simulink model "Battery_ConstT_Lumped"  (R2026b)
settings: Solver=VariableStepAuto
undefined symbols (not defined in the file or in its folder): battery_builder_rtmsupport, gcbh, Vehicle
libraries: Battery_ConstT_Lumped_lib x10
settings Model: Creator=andrei  LastModifiedBy=andrei

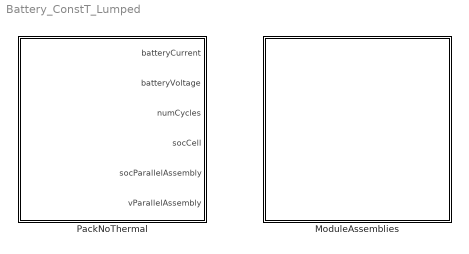
== system Battery_ConstT_Lumped ==
  ModuleAssemblies : Subsystem
  PackNoThermal : Subsystem  LoadFcn=battery_builder_rtmsupport('loadfcn',gcbh);  mask{BatteryPack=Vehicle.Powertrain.Power.Battery.BatteryPack}
      mask prompts: BatteryPack "Cell parameter structure (single-cell values)"
      mask help: Constant-temperature battery pack: 75 cells in series and 5 in parallel. Supply single-cell capacity (Ah), open-circuit voltage (V), resistance (Ohm), voltage limits, SOC and temperature lookup data. Series/parallel scaling is performed internally by the lumping adapters. Each module has one scalar representative-cell state.
      settings: CopyFcn=battery_builder_rtmsupport('copyfcn',gcbh);  PreCopyFcn=battery_builder_rtmsupport('precopyfcn',gcbh);  PreDeleteFcn=battery_builder_rtmsupport('predeletefcn',gcbh);  PortSchema="{\"entries\":[{\"content\":{\"sides\":[{\"content\":{\"connectorIds\":[\"LConn1\"]},\"type\":\"ConnectorPlacement.EquallySpacedRectSide\",\"uuid\":\"573f1e22-4fbd-4738-9df4-0664fa5945b1\"},{\"content\":{\"connectorIds\":[\"RConn1\"],\"side\":\"RIGHT\"},\"type\":\"ConnectorPlacement.EquallySpacedRectSide\",\"uuid\":\"3b7d0607-87fd-441c-83fa-686a76e2ac3c\"},{\"content\":{\"side\":\"TOP\"},\"type\":\"ConnectorPlacement.EquallySpacedRectSide\",\"uuid\":\"c7cf6d18-6b66-4f32-bb78-2b2f851634dd\"},{\"content\":{\"connectorIds\":[\"Out1\",\"Out2\",\"Out3\",\"Out4\",\"Out5\",\"Out6\"],\"side\":\"BOTTOM\"},\"type\":\"ConnectorPlacement.EquallySpacedRectSide\",\"uuid\":\"e3b01d7d-4c21-4d45-a142-ed30dadf23ae\"}]},\"type\":\"ConnectorPlacement.EquallySpacedConnector\",\"uuid\":\"ee102ac4-66a3-49fe-a4f4-6ac82dff7d13\"}],\"packageUris\":[\"http://schema.mathworks.com/mf0/Connector/R2020b\"],\"version\":\"1.0\"}"
      mask Display: image('$imagefile')

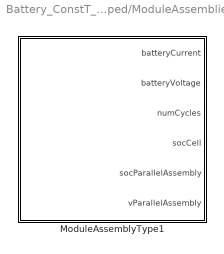
== system Battery_ConstT_Lumped/ModuleAssemblies ==
  ModuleAssemblyType1 : Subsystem  LoadFcn=battery_builder_rtmsupport('loadfcn',gcbh);
      settings: CopyFcn=battery_builder_rtmsupport('copyfcn',gcbh);  PreCopyFcn=battery_builder_rtmsupport('precopyfcn',gcbh);  PreDeleteFcn=battery_builder_rtmsupport('predeletefcn',gcbh);  PortSchema="{\"entries\":[{\"content\":{\"sides\":[{\"content\":{\"connectorIds\":[\"LConn1\"]},\"type\":\"ConnectorPlacement.EquallySpacedRectSide\",\"uuid\":\"573f1e22-4fbd-4738-9df4-0664fa5945b1\"},{\"content\":{\"connectorIds\":[\"RConn1\"],\"side\":\"RIGHT\"},\"type\":\"ConnectorPlacement.EquallySpacedRectSide\",\"uuid\":\"3b7d0607-87fd-441c-83fa-686a76e2ac3c\"},{\"content\":{\"side\":\"TOP\"},\"type\":\"ConnectorPlacement.EquallySpacedRectSide\",\"uuid\":\"c7cf6d18-6b66-4f32-bb78-2b2f851634dd\"},{\"content\":{\"connectorIds\":[\"Out1\",\"Out2\",\"Out3\",\"Out4\",\"Out5\",\"Out6\"],\"side\":\"BOTTOM\"},\"type\":\"ConnectorPlacement.EquallySpacedRectSide\",\"uuid\":\"1d9f9d4f-5931-4e62-be25-ddff82a8678d\"}]},\"type\":\"ConnectorPlacement.EquallySpacedConnector\",\"uuid\":\"ee102ac4-66a3-49fe-a4f4-6ac82dff7d13\"}],\"packageUris\":[\"http://schema.mathworks.com/mf0/Connector/R2020b\"],\"version\":\"1.0\"}"
      mask Display: image('$imagefile')

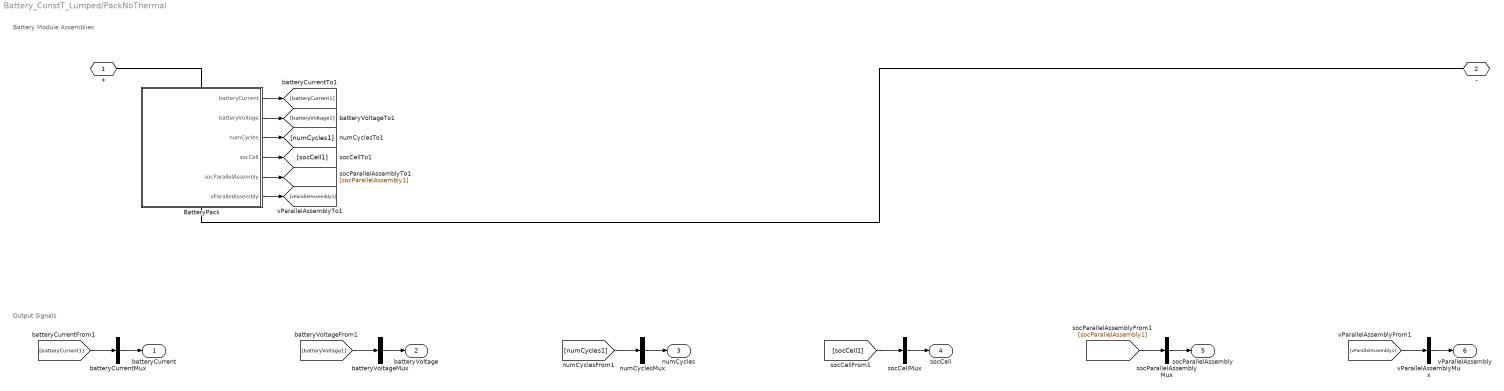
== system Battery_ConstT_Lumped/PackNoThermal ==
  note: Battery Module Assemblies
  note: Output Signals
  BatteryPack : Subsystem  LoadFcn=battery_builder_rtmsupport('loadfcn',gcbh);
      settings: CopyFcn=battery_builder_rtmsupport('copyfcn',gcbh);  PreCopyFcn=battery_builder_rtmsupport('precopyfcn',gcbh);  PreDeleteFcn=battery_builder_rtmsupport('predeletefcn',gcbh);  PortSchema="{\"entries\":[{\"content\":{\"sides\":[{\"content\":{\"connectorIds\":[\"LConn1\"]},\"type\":\"ConnectorPlacement.EquallySpacedRectSide\",\"uuid\":\"573f1e22-4fbd-4738-9df4-0664fa5945b1\"},{\"content\":{\"connectorIds\":[\"RConn1\"],\"side\":\"RIGHT\"},\"type\":\"ConnectorPlacement.EquallySpacedRectSide\",\"uuid\":\"3b7d0607-87fd-441c-83fa-686a76e2ac3c\"},{\"content\":{\"side\":\"TOP\"},\"type\":\"ConnectorPlacement.EquallySpacedRectSide\",\"uuid\":\"c7cf6d18-6b66-4f32-bb78-2b2f851634dd\"},{\"content\":{\"connectorIds\":[\"Out1\",\"Out2\",\"Out3\",\"Out4\",\"Out5\",\"Out6\"],\"side\":\"BOTTOM\"},\"type\":\"ConnectorPlacement.EquallySpacedRectSide\",\"uuid\":\"1d9f9d4f-5931-4e62-be25-ddff82a8678d\"}]},\"type\":\"ConnectorPlacement.EquallySpacedConnector\",\"uuid\":\"ee102ac4-66a3-49fe-a4f4-6ac82dff7d13\"}],\"packageUris\":[\"http://schema.mathworks.com/mf0/Connector/R2020b\"],\"version\":\"1.0\"}"
      mask Display: image('$imagefile')
  batteryCurrentMux : Mux  Inputs=1
  batteryVoltageMux : Mux  Inputs=1
  numCyclesMux : Mux  Inputs=1
  socCellMux : Mux  Inputs=1
  socParallelAssemblyMux : Mux  Inputs=1
  vParallelAssemblyMux : Mux  Inputs=1
  + : PMIOPort  Side=Left
  - : PMIOPort  Port=2  Side=Right
  batteryCurrent : Outport
  batteryVoltage : Outport  Port=2
  numCycles : Outport  Port=3
  socCell : Outport  Port=4
  socParallelAssembly : Outport  Port=5
  vParallelAssembly : Outport  Port=6
  wires:
  BatteryPack/1(batteryCurrent) -> [batteryCurrent1]
  batteryCurrentMux/1 -> batteryCurrent/1
  [batteryCurrent1] -> batteryCurrentMux/1
  BatteryPack/2(batteryVoltage) -> [batteryVoltage1]
  batteryVoltageMux/1 -> batteryVoltage/1
  [batteryVoltage1] -> batteryVoltageMux/1
  BatteryPack/3(numCycles) -> [numCycles1]
  numCyclesMux/1 -> numCycles/1
  [numCycles1] -> numCyclesMux/1
  BatteryPack/4(socCell) -> [socCell1]
  socCellMux/1 -> socCell/1
  [socCell1] -> socCellMux/1
  BatteryPack/5(socParallelAssembly) -> [socParallelAssembly1]
  socParallelAssemblyMux/1 -> socParallelAssembly/1
  [socParallelAssembly1] -> socParallelAssemblyMux/1
  BatteryPack/6(vParallelAssembly) -> [vParallelAssembly1]
  vParallelAssemblyMux/1 -> vParallelAssembly/1
  [vParallelAssembly1] -> vParallelAssemblyMux/1
  connections:
  BatteryPack/LConn1 -- +/RConn1
  BatteryPack/RConn1 -- -/RConn1

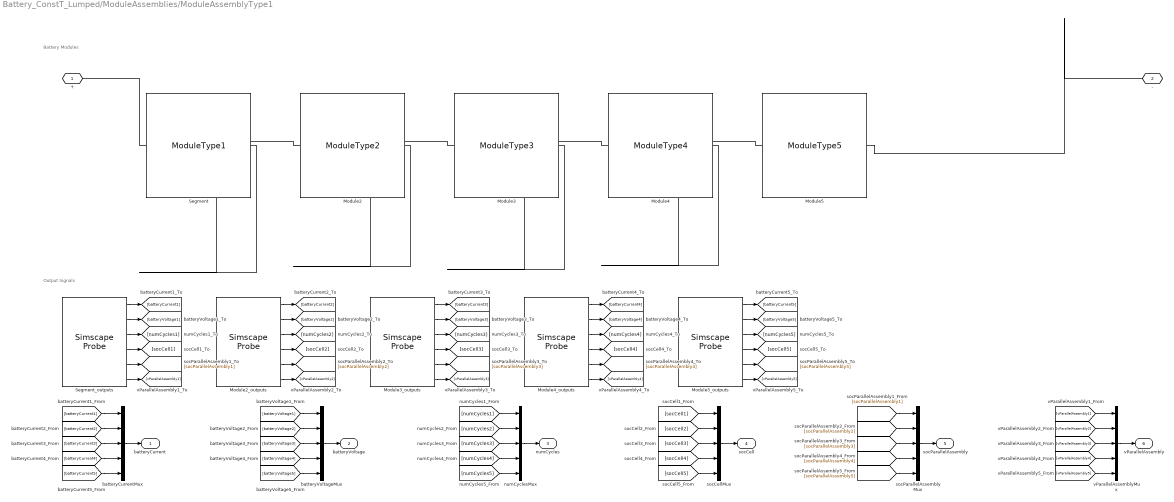
== system Battery_ConstT_Lumped/ModuleAssemblies/ModuleAssemblyType1 ==
  note: Battery Modules
  note: Output Signals
  Module2 : Battery_ConstT_Lumped_lib/Modules/ModuleType2  BatteryCapacityCell=27 A*hr  ExtrapolationMethodCell=simscape.enum.extrapolation.nearest  SOCBreakpointsCell=[0, .1, .25, .5, .75, .9, 1]  TemperatureBreakpointsCell=[278, 293, 313] K  OpenCircuitVoltageThermalCell=[3.49, 3.5, 3.51; 3.55, 3.57, 3.56; 3.62, 3.63, 3.64; 3.71, 3.71, 3.72; 3.91, 3.93, 3.94; 4.07, 4.08, 4.08; 4.19, 4.19, 4.19] V  VoltageRangeCell=[0, inf] V  ResistanceSOCBreakpointsCell=[0, .1, .25, .5, .75, .9, 1]  ResistanceTemperatureBreakpointsCell=[278, 293, 313] K  R0ThermalCell=[.0117, .0085, .009; .011, .0085, .009; .0114, .0087, .0092; .0107, .0082, .0088; .0107, .0083, .0091; .0113, .0085, .0089; .0116, .0085, .0089] Ohm  SimulationTemperatureCell=298.15 K  socCell_specify=off  socCell_priority=High  socCell=1  socCell_nominal_specify=off  socCell_nominal_value=1  socCell_nominal_unit=1  batteryVoltage_specify=off  batteryVoltage_priority=None  batteryVoltage=0 V  batteryVoltage_nominal_specify=off  batteryVoltage_nominal_value=1  batteryVoltage_nominal_unit=V  batteryCurrent_specify=off  batteryCurrent_priority=None  batteryCurrent=0 A  batteryCurrent_nominal_specify=off  batteryCurrent_nominal_value=1  batteryCurrent_nominal_unit=A  numCycles_specify=off  numCycles_priority=High  numCycles=0  numCycles_nominal_specify=off  numCycles_nominal_value=1  numCycles_nominal_unit=1  vParallelAssembly_specify=off  vParallelAssembly_priority=None  vParallelAssembly=repmat(0, 15, 1) V  vParallelAssembly_nominal_specify=off  vParallelAssembly_nominal_value=1  vParallelAssembly_nominal_unit=V  socParallelAssembly_specify=off  socParallelAssembly_priority=None  socParallelAssembly=repmat(1, 15, 1)  socParallelAssembly_nominal_specify=off  socParallelAssembly_nominal_value=1  socParallelAssembly_nominal_unit=1
  Module2_outputs : SimscapeProbe  BoundBlock=4  Variables="{\"batteryCurrent\":{\"Probing\":\"ON\"},\"batteryVoltage\":{\"Probing\":\"ON\"},\"numCycles\":{\"Probing\":\"ON\"},\"socCell\":{\"Probing\":\"ON\"},\"socParallelAssembly\":{\"Probing\":\"ON\"},\"vParallelAssembly\":{\"Probing\":\"ON\"}}"
  Module3 : Battery_ConstT_Lumped_lib/Modules/ModuleType3  BatteryCapacityCell=27 A*hr  ExtrapolationMethodCell=simscape.enum.extrapolation.nearest  SOCBreakpointsCell=[0, .1, .25, .5, .75, .9, 1]  TemperatureBreakpointsCell=[278, 293, 313] K  OpenCircuitVoltageThermalCell=[3.49, 3.5, 3.51; 3.55, 3.57, 3.56; 3.62, 3.63, 3.64; 3.71, 3.71, 3.72; 3.91, 3.93, 3.94; 4.07, 4.08, 4.08; 4.19, 4.19, 4.19] V  VoltageRangeCell=[0, inf] V  ResistanceSOCBreakpointsCell=[0, .1, .25, .5, .75, .9, 1]  ResistanceTemperatureBreakpointsCell=[278, 293, 313] K  R0ThermalCell=[.0117, .0085, .009; .011, .0085, .009; .0114, .0087, .0092; .0107, .0082, .0088; .0107, .0083, .0091; .0113, .0085, .0089; .0116, .0085, .0089] Ohm  SimulationTemperatureCell=298.15 K  socCell_specify=off  socCell_priority=High  socCell=1  socCell_nominal_specify=off  socCell_nominal_value=1  socCell_nominal_unit=1  batteryVoltage_specify=off  batteryVoltage_priority=None  batteryVoltage=0 V  batteryVoltage_nominal_specify=off  batteryVoltage_nominal_value=1  batteryVoltage_nominal_unit=V  batteryCurrent_specify=off  batteryCurrent_priority=None  batteryCurrent=0 A  batteryCurrent_nominal_specify=off  batteryCurrent_nominal_value=1  batteryCurrent_nominal_unit=A  numCycles_specify=off  numCycles_priority=High  numCycles=0  numCycles_nominal_specify=off  numCycles_nominal_value=1  numCycles_nominal_unit=1  vParallelAssembly_specify=off  vParallelAssembly_priority=None  vParallelAssembly=repmat(0, 15, 1) V  vParallelAssembly_nominal_specify=off  vParallelAssembly_nominal_value=1  vParallelAssembly_nominal_unit=V  socParallelAssembly_specify=off  socParallelAssembly_priority=None  socParallelAssembly=repmat(1, 15, 1)  socParallelAssembly_nominal_specify=off  socParallelAssembly_nominal_value=1  socParallelAssembly_nominal_unit=1
  Module3_outputs : SimscapeProbe  BoundBlock=5  Variables="{\"batteryCurrent\":{\"Probing\":\"ON\"},\"batteryVoltage\":{\"Probing\":\"ON\"},\"numCycles\":{\"Probing\":\"ON\"},\"socCell\":{\"Probing\":\"ON\"},\"socParallelAssembly\":{\"Probing\":\"ON\"},\"vParallelAssembly\":{\"Probing\":\"ON\"}}"
  Module4 : Battery_ConstT_Lumped_lib/Modules/ModuleType4  BatteryCapacityCell=27 A*hr  ExtrapolationMethodCell=simscape.enum.extrapolation.nearest  SOCBreakpointsCell=[0, .1, .25, .5, .75, .9, 1]  TemperatureBreakpointsCell=[278, 293, 313] K  OpenCircuitVoltageThermalCell=[3.49, 3.5, 3.51; 3.55, 3.57, 3.56; 3.62, 3.63, 3.64; 3.71, 3.71, 3.72; 3.91, 3.93, 3.94; 4.07, 4.08, 4.08; 4.19, 4.19, 4.19] V  VoltageRangeCell=[0, inf] V  ResistanceSOCBreakpointsCell=[0, .1, .25, .5, .75, .9, 1]  ResistanceTemperatureBreakpointsCell=[278, 293, 313] K  R0ThermalCell=[.0117, .0085, .009; .011, .0085, .009; .0114, .0087, .0092; .0107, .0082, .0088; .0107, .0083, .0091; .0113, .0085, .0089; .0116, .0085, .0089] Ohm  SimulationTemperatureCell=298.15 K  socCell_specify=off  socCell_priority=High  socCell=1  socCell_nominal_specify=off  socCell_nominal_value=1  socCell_nominal_unit=1  batteryVoltage_specify=off  batteryVoltage_priority=None  batteryVoltage=0 V  batteryVoltage_nominal_specify=off  batteryVoltage_nominal_value=1  batteryVoltage_nominal_unit=V  batteryCurrent_specify=off  batteryCurrent_priority=None  batteryCurrent=0 A  batteryCurrent_nominal_specify=off  batteryCurrent_nominal_value=1  batteryCurrent_nominal_unit=A  numCycles_specify=off  numCycles_priority=High  numCycles=0  numCycles_nominal_specify=off  numCycles_nominal_value=1  numCycles_nominal_unit=1  vParallelAssembly_specify=off  vParallelAssembly_priority=None  vParallelAssembly=repmat(0, 15, 1) V  vParallelAssembly_nominal_specify=off  vParallelAssembly_nominal_value=1  vParallelAssembly_nominal_unit=V  socParallelAssembly_specify=off  socParallelAssembly_priority=None  socParallelAssembly=repmat(1, 15, 1)  socParallelAssembly_nominal_specify=off  socParallelAssembly_nominal_value=1  socParallelAssembly_nominal_unit=1
  Module4_outputs : SimscapeProbe  BoundBlock=6  Variables="{\"batteryCurrent\":{\"Probing\":\"ON\"},\"batteryVoltage\":{\"Probing\":\"ON\"},\"numCycles\":{\"Probing\":\"ON\"},\"socCell\":{\"Probing\":\"ON\"},\"socParallelAssembly\":{\"Probing\":\"ON\"},\"vParallelAssembly\":{\"Probing\":\"ON\"}}"
  Module5 : Battery_ConstT_Lumped_lib/Modules/ModuleType5  BatteryCapacityCell=27 A*hr  ExtrapolationMethodCell=simscape.enum.extrapolation.nearest  SOCBreakpointsCell=[0, .1, .25, .5, .75, .9, 1]  TemperatureBreakpointsCell=[278, 293, 313] K  OpenCircuitVoltageThermalCell=[3.49, 3.5, 3.51; 3.55, 3.57, 3.56; 3.62, 3.63, 3.64; 3.71, 3.71, 3.72; 3.91, 3.93, 3.94; 4.07, 4.08, 4.08; 4.19, 4.19, 4.19] V  VoltageRangeCell=[0, inf] V  ResistanceSOCBreakpointsCell=[0, .1, .25, .5, .75, .9, 1]  ResistanceTemperatureBreakpointsCell=[278, 293, 313] K  R0ThermalCell=[.0117, .0085, .009; .011, .0085, .009; .0114, .0087, .0092; .0107, .0082, .0088; .0107, .0083, .0091; .0113, .0085, .0089; .0116, .0085, .0089] Ohm  SimulationTemperatureCell=298.15 K  socCell_specify=off  socCell_priority=High  socCell=1  socCell_nominal_specify=off  socCell_nominal_value=1  socCell_nominal_unit=1  batteryVoltage_specify=off  batteryVoltage_priority=None  batteryVoltage=0 V  batteryVoltage_nominal_specify=off  batteryVoltage_nominal_value=1  batteryVoltage_nominal_unit=V  batteryCurrent_specify=off  batteryCurrent_priority=None  batteryCurrent=0 A  batteryCurrent_nominal_specify=off  batteryCurrent_nominal_value=1  batteryCurrent_nominal_unit=A  numCycles_specify=off  numCycles_priority=High  numCycles=0  numCycles_nominal_specify=off  numCycles_nominal_value=1  numCycles_nominal_unit=1  vParallelAssembly_specify=off  vParallelAssembly_priority=None  vParallelAssembly=repmat(0, 15, 1) V  vParallelAssembly_nominal_specify=off  vParallelAssembly_nominal_value=1  vParallelAssembly_nominal_unit=V  socParallelAssembly_specify=off  socParallelAssembly_priority=None  socParallelAssembly=repmat(1, 15, 1)  socParallelAssembly_nominal_specify=off  socParallelAssembly_nominal_value=1  socParallelAssembly_nominal_unit=1
  Module5_outputs : SimscapeProbe  BoundBlock=7  Variables="{\"batteryCurrent\":{\"Probing\":\"ON\"},\"batteryVoltage\":{\"Probing\":\"ON\"},\"numCycles\":{\"Probing\":\"ON\"},\"socCell\":{\"Probing\":\"ON\"},\"socParallelAssembly\":{\"Probing\":\"ON\"},\"vParallelAssembly\":{\"Probing\":\"ON\"}}"
  Segment : Battery_ConstT_Lumped_lib/Modules/ModuleType1  BatteryCapacityCell=27 A*hr  ExtrapolationMethodCell=simscape.enum.extrapolation.nearest  SOCBreakpointsCell=[0, .1, .25, .5, .75, .9, 1]  TemperatureBreakpointsCell=[278, 293, 313] K  OpenCircuitVoltageThermalCell=[3.49, 3.5, 3.51; 3.55, 3.57, 3.56; 3.62, 3.63, 3.64; 3.71, 3.71, 3.72; 3.91, 3.93, 3.94; 4.07, 4.08, 4.08; 4.19, 4.19, 4.19] V  VoltageRangeCell=[0, inf] V  ResistanceSOCBreakpointsCell=[0, .1, .25, .5, .75, .9, 1]  ResistanceTemperatureBreakpointsCell=[278, 293, 313] K  R0ThermalCell=[.0117, .0085, .009; .011, .0085, .009; .0114, .0087, .0092; .0107, .0082, .0088; .0107, .0083, .0091; .0113, .0085, .0089; .0116, .0085, .0089] Ohm  SimulationTemperatureCell=298.15 K  socCell_specify=off  socCell_priority=High  socCell=1  socCell_nominal_specify=off  socCell_nominal_value=1  socCell_nominal_unit=1  batteryVoltage_specify=off  batteryVoltage_priority=None  batteryVoltage=0 V  batteryVoltage_nominal_specify=off  batteryVoltage_nominal_value=1  batteryVoltage_nominal_unit=V  batteryCurrent_specify=off  batteryCurrent_priority=None  batteryCurrent=0 A  batteryCurrent_nominal_specify=off  batteryCurrent_nominal_value=1  batteryCurrent_nominal_unit=A  numCycles_specify=off  numCycles_priority=High  numCycles=0  numCycles_nominal_specify=off  numCycles_nominal_value=1  numCycles_nominal_unit=1  vParallelAssembly_specify=off  vParallelAssembly_priority=None  vParallelAssembly=repmat(0, 15, 1) V  vParallelAssembly_nominal_specify=off  vParallelAssembly_nominal_value=1  vParallelAssembly_nominal_unit=V  socParallelAssembly_specify=off  socParallelAssembly_priority=None  socParallelAssembly=repmat(1, 15, 1)  socParallelAssembly_nominal_specify=off  socParallelAssembly_nominal_value=1  socParallelAssembly_nominal_unit=1
  Segment_outputs : SimscapeProbe  BoundBlock=3  Variables="{\"batteryCurrent\":{\"Probing\":\"ON\"},\"batteryVoltage\":{\"Probing\":\"ON\"},\"numCycles\":{\"Probing\":\"ON\"},\"socCell\":{\"Probing\":\"ON\"},\"socParallelAssembly\":{\"Probing\":\"ON\"},\"vParallelAssembly\":{\"Probing\":\"ON\"}}"
  batteryCurrentMux : Mux  Inputs=5
  batteryVoltageMux : Mux  Inputs=5
  numCyclesMux : Mux  Inputs=5
  socCellMux : Mux  Inputs=5
  socParallelAssemblyMux : Mux  Inputs=5
  vParallelAssemblyMux : Mux  Inputs=5
  + : PMIOPort  Side=Left
  - : PMIOPort  Port=2  Side=Right
  batteryCurrent : Outport
  batteryVoltage : Outport  Port=2
  numCycles : Outport  Port=3
  socCell : Outport  Port=4
  socParallelAssembly : Outport  Port=5
  vParallelAssembly : Outport  Port=6
  wires:
  Segment_outputs/1 -> [batteryCurrent1]
  batteryCurrentMux/1 -> batteryCurrent/1
  [batteryCurrent1] -> batteryCurrentMux/1
  Segment_outputs/2 -> [batteryVoltage1]
  batteryVoltageMux/1 -> batteryVoltage/1
  [batteryVoltage1] -> batteryVoltageMux/1
  Segment_outputs/3 -> [numCycles1]
  numCyclesMux/1 -> numCycles/1
  [numCycles1] -> numCyclesMux/1
  Segment_outputs/4 -> [socCell1]
  socCellMux/1 -> socCell/1
  [socCell1] -> socCellMux/1
  Segment_outputs/5 -> [socParallelAssembly1]
  socParallelAssemblyMux/1 -> socParallelAssembly/1
  [socParallelAssembly1] -> socParallelAssemblyMux/1
  Segment_outputs/6 -> [vParallelAssembly1]
  vParallelAssemblyMux/1 -> vParallelAssembly/1
  [vParallelAssembly1] -> vParallelAssemblyMux/1
  Module2_outputs/1 -> [batteryCurrent2]
  [batteryCurrent2] -> batteryCurrentMux/2
  Module2_outputs/2 -> [batteryVoltage2]
  [batteryVoltage2] -> batteryVoltageMux/2
  Module2_outputs/3 -> [numCycles2]
  [numCycles2] -> numCyclesMux/2
  Module2_outputs/4 -> [socCell2]
  [socCell2] -> socCellMux/2
  Module2_outputs/5 -> [socParallelAssembly2]
  [socParallelAssembly2] -> socParallelAssemblyMux/2
  Module2_outputs/6 -> [vParallelAssembly2]
  [vParallelAssembly2] -> vParallelAssemblyMux/2
  Module3_outputs/1 -> [batteryCurrent3]
  [batteryCurrent3] -> batteryCurrentMux/3
  Module3_outputs/2 -> [batteryVoltage3]
  [batteryVoltage3] -> batteryVoltageMux/3
  Module3_outputs/3 -> [numCycles3]
  [numCycles3] -> numCyclesMux/3
  Module3_outputs/4 -> [socCell3]
  [socCell3] -> socCellMux/3
  Module3_outputs/5 -> [socParallelAssembly3]
  [socParallelAssembly3] -> socParallelAssemblyMux/3
  Module3_outputs/6 -> [vParallelAssembly3]
  [vParallelAssembly3] -> vParallelAssemblyMux/3
  Module4_outputs/1 -> [batteryCurrent4]
  [batteryCurrent4] -> batteryCurrentMux/4
  Module4_outputs/2 -> [batteryVoltage4]
  [batteryVoltage4] -> batteryVoltageMux/4
  Module4_outputs/3 -> [numCycles4]
  [numCycles4] -> numCyclesMux/4
  Module4_outputs/4 -> [socCell4]
  [socCell4] -> socCellMux/4
  Module4_outputs/5 -> [socParallelAssembly4]
  [socParallelAssembly4] -> socParallelAssemblyMux/4
  Module4_outputs/6 -> [vParallelAssembly4]
  [vParallelAssembly4] -> vParallelAssemblyMux/4
  Module5_outputs/1 -> [batteryCurrent5]
  [batteryCurrent5] -> batteryCurrentMux/5
  Module5_outputs/2 -> [batteryVoltage5]
  [batteryVoltage5] -> batteryVoltageMux/5
  Module5_outputs/3 -> [numCycles5]
  [numCycles5] -> numCyclesMux/5
  Module5_outputs/4 -> [socCell5]
  [socCell5] -> socCellMux/5
  Module5_outputs/5 -> [socParallelAssembly5]
  [socParallelAssembly5] -> socParallelAssemblyMux/5
  Module5_outputs/6 -> [vParallelAssembly5]
  [vParallelAssembly5] -> vParallelAssemblyMux/5
  connections:
  Module2/LConn1 -- Segment/RConn1
  Module3/LConn1 -- Module2/RConn1
  Module4/LConn1 -- Module3/RConn1
  Module5/LConn1 -- Module4/RConn1
  Segment/LConn1 -- +/RConn1
  Module5/RConn1 -- -/RConn1

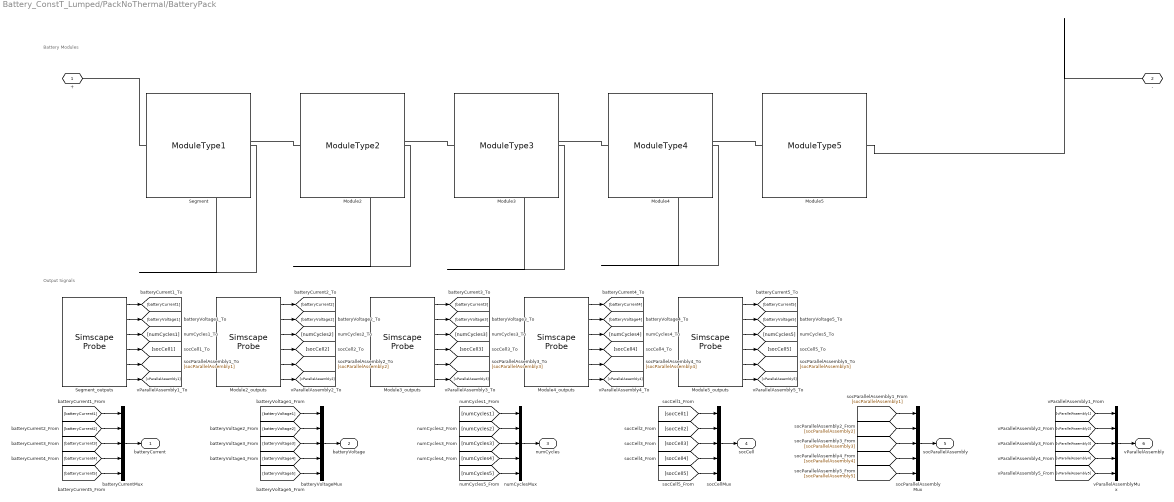
== system Battery_ConstT_Lumped/PackNoThermal/BatteryPack ==
  note: Output Signals
  note: Battery Modules
  Module2 : Battery_ConstT_Lumped_lib/Modules/ModuleType2  BatteryCapacityCell=BatteryPack.BatteryCapacityCell.Value A*hr  ExtrapolationMethodCell=simscape.enum.extrapolation.nearest  SOCBreakpointsCell=BatteryPack.SOCBreakpointsCell.Value  TemperatureBreakpointsCell=BatteryPack.TemperatureBreakpointsCell.Value K  OpenCircuitVoltageThermalCell=BatteryPack.OpenCircuitVoltageThermalCell.Value V  VoltageRangeCell=BatteryPack.VoltageRangeCell.Value V  ResistanceSOCBreakpointsCell=BatteryPack.ResistanceSOCBreakpointsCell.Value  ResistanceTemperatureBreakpointsCell=BatteryPack.ResistanceTemperatureBreakpointsCell.Value K  R0ThermalCell=BatteryPack.R0ThermalCell.Value Ohm  SimulationTemperatureCell=BatteryPack.SimulationTemperatureCell.Value K  socCell_specify=on  socCell_priority=High  socCell=BatteryPack.SOCInit.Value  socCell_nominal_specify=off  socCell_nominal_value=1  socCell_nominal_unit=1  batteryVoltage_specify=off  batteryVoltage_priority=None  batteryVoltage=0 V  batteryVoltage_nominal_specify=off  batteryVoltage_nominal_value=1  batteryVoltage_nominal_unit=V  batteryCurrent_specify=off  batteryCurrent_priority=None  batteryCurrent=0 A  batteryCurrent_nominal_specify=off  batteryCurrent_nominal_value=1  batteryCurrent_nominal_unit=A  numCycles_specify=off  numCycles_priority=High  numCycles=0  numCycles_nominal_specify=off  numCycles_nominal_value=1  numCycles_nominal_unit=1  vParallelAssembly_specify=off  vParallelAssembly_priority=None  vParallelAssembly=repmat(0, 15, 1) V  vParallelAssembly_nominal_specify=off  vParallelAssembly_nominal_value=1  vParallelAssembly_nominal_unit=V  socParallelAssembly_specify=off  socParallelAssembly_priority=None  socParallelAssembly=repmat(1, 15, 1)  socParallelAssembly_nominal_specify=off  socParallelAssembly_nominal_value=1  socParallelAssembly_nominal_unit=1
  Module2_outputs : SimscapeProbe  BoundBlock=91  Variables="{\"batteryCurrent\":{\"Probing\":\"ON\"},\"batteryVoltage\":{\"Probing\":\"ON\"},\"numCycles\":{\"Probing\":\"ON\"},\"socCell\":{\"Probing\":\"ON\"},\"socParallelAssembly\":{\"Probing\":\"ON\"},\"vParallelAssembly\":{\"Probing\":\"ON\"}}"
  Module3 : Battery_ConstT_Lumped_lib/Modules/ModuleType3  BatteryCapacityCell=BatteryPack.BatteryCapacityCell.Value A*hr  ExtrapolationMethodCell=simscape.enum.extrapolation.nearest  SOCBreakpointsCell=BatteryPack.SOCBreakpointsCell.Value  TemperatureBreakpointsCell=BatteryPack.TemperatureBreakpointsCell.Value K  OpenCircuitVoltageThermalCell=BatteryPack.OpenCircuitVoltageThermalCell.Value V  VoltageRangeCell=BatteryPack.VoltageRangeCell.Value V  ResistanceSOCBreakpointsCell=BatteryPack.ResistanceSOCBreakpointsCell.Value  ResistanceTemperatureBreakpointsCell=BatteryPack.ResistanceTemperatureBreakpointsCell.Value K  R0ThermalCell=BatteryPack.R0ThermalCell.Value Ohm  SimulationTemperatureCell=BatteryPack.SimulationTemperatureCell.Value K  socCell_specify=on  socCell_priority=High  socCell=BatteryPack.SOCInit.Value  socCell_nominal_specify=off  socCell_nominal_value=1  socCell_nominal_unit=1  batteryVoltage_specify=off  batteryVoltage_priority=None  batteryVoltage=0 V  batteryVoltage_nominal_specify=off  batteryVoltage_nominal_value=1  batteryVoltage_nominal_unit=V  batteryCurrent_specify=off  batteryCurrent_priority=None  batteryCurrent=0 A  batteryCurrent_nominal_specify=off  batteryCurrent_nominal_value=1  batteryCurrent_nominal_unit=A  numCycles_specify=off  numCycles_priority=High  numCycles=0  numCycles_nominal_specify=off  numCycles_nominal_value=1  numCycles_nominal_unit=1  vParallelAssembly_specify=off  vParallelAssembly_priority=None  vParallelAssembly=repmat(0, 15, 1) V  vParallelAssembly_nominal_specify=off  vParallelAssembly_nominal_value=1  vParallelAssembly_nominal_unit=V  socParallelAssembly_specify=off  socParallelAssembly_priority=None  socParallelAssembly=repmat(1, 15, 1)  socParallelAssembly_nominal_specify=off  socParallelAssembly_nominal_value=1  socParallelAssembly_nominal_unit=1
  Module3_outputs : SimscapeProbe  BoundBlock=93  Variables="{\"batteryCurrent\":{\"Probing\":\"ON\"},\"batteryVoltage\":{\"Probing\":\"ON\"},\"numCycles\":{\"Probing\":\"ON\"},\"socCell\":{\"Probing\":\"ON\"},\"socParallelAssembly\":{\"Probing\":\"ON\"},\"vParallelAssembly\":{\"Probing\":\"ON\"}}"
  Module4 : Battery_ConstT_Lumped_lib/Modules/ModuleType4  BatteryCapacityCell=BatteryPack.BatteryCapacityCell.Value A*hr  ExtrapolationMethodCell=simscape.enum.extrapolation.nearest  SOCBreakpointsCell=BatteryPack.SOCBreakpointsCell.Value  TemperatureBreakpointsCell=BatteryPack.TemperatureBreakpointsCell.Value K  OpenCircuitVoltageThermalCell=BatteryPack.OpenCircuitVoltageThermalCell.Value V  VoltageRangeCell=BatteryPack.VoltageRangeCell.Value V  ResistanceSOCBreakpointsCell=BatteryPack.ResistanceSOCBreakpointsCell.Value  ResistanceTemperatureBreakpointsCell=BatteryPack.ResistanceTemperatureBreakpointsCell.Value K  R0ThermalCell=BatteryPack.R0ThermalCell.Value Ohm  SimulationTemperatureCell=BatteryPack.SimulationTemperatureCell.Value K  socCell_specify=on  socCell_priority=High  socCell=BatteryPack.SOCInit.Value  socCell_nominal_specify=off  socCell_nominal_value=1  socCell_nominal_unit=1  batteryVoltage_specify=off  batteryVoltage_priority=None  batteryVoltage=0 V  batteryVoltage_nominal_specify=off  batteryVoltage_nominal_value=1  batteryVoltage_nominal_unit=V  batteryCurrent_specify=off  batteryCurrent_priority=None  batteryCurrent=0 A  batteryCurrent_nominal_specify=off  batteryCurrent_nominal_value=1  batteryCurrent_nominal_unit=A  numCycles_specify=off  numCycles_priority=High  numCycles=0  numCycles_nominal_specify=off  numCycles_nominal_value=1  numCycles_nominal_unit=1  vParallelAssembly_specify=off  vParallelAssembly_priority=None  vParallelAssembly=repmat(0, 15, 1) V  vParallelAssembly_nominal_specify=off  vParallelAssembly_nominal_value=1  vParallelAssembly_nominal_unit=V  socParallelAssembly_specify=off  socParallelAssembly_priority=None  socParallelAssembly=repmat(1, 15, 1)  socParallelAssembly_nominal_specify=off  socParallelAssembly_nominal_value=1  socParallelAssembly_nominal_unit=1
  Module4_outputs : SimscapeProbe  BoundBlock=95  Variables="{\"batteryCurrent\":{\"Probing\":\"ON\"},\"batteryVoltage\":{\"Probing\":\"ON\"},\"numCycles\":{\"Probing\":\"ON\"},\"socCell\":{\"Probing\":\"ON\"},\"socParallelAssembly\":{\"Probing\":\"ON\"},\"vParallelAssembly\":{\"Probing\":\"ON\"}}"
  Module5 : Battery_ConstT_Lumped_lib/Modules/ModuleType5  BatteryCapacityCell=BatteryPack.BatteryCapacityCell.Value A*hr  ExtrapolationMethodCell=simscape.enum.extrapolation.nearest  SOCBreakpointsCell=BatteryPack.SOCBreakpointsCell.Value  TemperatureBreakpointsCell=BatteryPack.TemperatureBreakpointsCell.Value K  OpenCircuitVoltageThermalCell=BatteryPack.OpenCircuitVoltageThermalCell.Value V  VoltageRangeCell=BatteryPack.VoltageRangeCell.Value V  ResistanceSOCBreakpointsCell=BatteryPack.ResistanceSOCBreakpointsCell.Value  ResistanceTemperatureBreakpointsCell=BatteryPack.ResistanceTemperatureBreakpointsCell.Value K  R0ThermalCell=BatteryPack.R0ThermalCell.Value Ohm  SimulationTemperatureCell=BatteryPack.SimulationTemperatureCell.Value K  socCell_specify=on  socCell_priority=High  socCell=BatteryPack.SOCInit.Value  socCell_nominal_specify=off  socCell_nominal_value=1  socCell_nominal_unit=1  batteryVoltage_specify=off  batteryVoltage_priority=None  batteryVoltage=0 V  batteryVoltage_nominal_specify=off  batteryVoltage_nominal_value=1  batteryVoltage_nominal_unit=V  batteryCurrent_specify=off  batteryCurrent_priority=None  batteryCurrent=0 A  batteryCurrent_nominal_specify=off  batteryCurrent_nominal_value=1  batteryCurrent_nominal_unit=A  numCycles_specify=off  numCycles_priority=High  numCycles=0  numCycles_nominal_specify=off  numCycles_nominal_value=1  numCycles_nominal_unit=1  vParallelAssembly_specify=off  vParallelAssembly_priority=None  vParallelAssembly=repmat(0, 15, 1) V  vParallelAssembly_nominal_specify=off  vParallelAssembly_nominal_value=1  vParallelAssembly_nominal_unit=V  socParallelAssembly_specify=off  socParallelAssembly_priority=None  socParallelAssembly=repmat(1, 15, 1)  socParallelAssembly_nominal_specify=off  socParallelAssembly_nominal_value=1  socParallelAssembly_nominal_unit=1
  Module5_outputs : SimscapeProbe  BoundBlock=97  Variables="{\"batteryCurrent\":{\"Probing\":\"ON\"},\"batteryVoltage\":{\"Probing\":\"ON\"},\"numCycles\":{\"Probing\":\"ON\"},\"socCell\":{\"Probing\":\"ON\"},\"socParallelAssembly\":{\"Probing\":\"ON\"},\"vParallelAssembly\":{\"Probing\":\"ON\"}}"
  Segment : Battery_ConstT_Lumped_lib/Modules/ModuleType1  BatteryCapacityCell=BatteryPack.BatteryCapacityCell.Value A*hr  ExtrapolationMethodCell=simscape.enum.extrapolation.nearest  SOCBreakpointsCell=BatteryPack.SOCBreakpointsCell.Value  TemperatureBreakpointsCell=BatteryPack.TemperatureBreakpointsCell.Value K  OpenCircuitVoltageThermalCell=BatteryPack.OpenCircuitVoltageThermalCell.Value V  VoltageRangeCell=BatteryPack.VoltageRangeCell.Value V  ResistanceSOCBreakpointsCell=BatteryPack.ResistanceSOCBreakpointsCell.Value  ResistanceTemperatureBreakpointsCell=BatteryPack.ResistanceTemperatureBreakpointsCell.Value K  R0ThermalCell=BatteryPack.R0ThermalCell.Value Ohm  SimulationTemperatureCell=BatteryPack.SimulationTemperatureCell.Value K  socCell_specify=on  socCell_priority=High  socCell=BatteryPack.SOCInit.Value  socCell_nominal_specify=off  socCell_nominal_value=1  socCell_nominal_unit=1  batteryVoltage_specify=off  batteryVoltage_priority=None  batteryVoltage=0 V  batteryVoltage_nominal_specify=off  batteryVoltage_nominal_value=1  batteryVoltage_nominal_unit=V  batteryCurrent_specify=off  batteryCurrent_priority=None  batteryCurrent=0 A  batteryCurrent_nominal_specify=off  batteryCurrent_nominal_value=1  batteryCurrent_nominal_unit=A  numCycles_specify=off  numCycles_priority=High  numCycles=0  numCycles_nominal_specify=off  numCycles_nominal_value=1  numCycles_nominal_unit=1  vParallelAssembly_specify=off  vParallelAssembly_priority=None  vParallelAssembly=repmat(0, 15, 1) V  vParallelAssembly_nominal_specify=off  vParallelAssembly_nominal_value=1  vParallelAssembly_nominal_unit=V  socParallelAssembly_specify=off  socParallelAssembly_priority=None  socParallelAssembly=repmat(1, 15, 1)  socParallelAssembly_nominal_specify=off  socParallelAssembly_nominal_value=1  socParallelAssembly_nominal_unit=1
  Segment_outputs : SimscapeProbe  BoundBlock=99  Variables="{\"batteryCurrent\":{\"Probing\":\"ON\"},\"batteryVoltage\":{\"Probing\":\"ON\"},\"numCycles\":{\"Probing\":\"ON\"},\"socCell\":{\"Probing\":\"ON\"},\"socParallelAssembly\":{\"Probing\":\"ON\"},\"vParallelAssembly\":{\"Probing\":\"ON\"}}"
  batteryCurrentMux : Mux  Inputs=5
  batteryVoltageMux : Mux  Inputs=5
  numCyclesMux : Mux  Inputs=5
  socCellMux : Mux  Inputs=5
  socParallelAssemblyMux : Mux  Inputs=5
  vParallelAssemblyMux : Mux  Inputs=5
  + : PMIOPort  Side=Left
  - : PMIOPort  Port=2  Side=Right
  batteryCurrent : Outport
  batteryVoltage : Outport  Port=2
  numCycles : Outport  Port=3
  socCell : Outport  Port=4
  socParallelAssembly : Outport  Port=5
  vParallelAssembly : Outport  Port=6
  wires:
  [vParallelAssembly5] -> vParallelAssemblyMux/5
  Module5_outputs/6 -> [vParallelAssembly5]
  [socParallelAssembly5] -> socParallelAssemblyMux/5
  Module5_outputs/5 -> [socParallelAssembly5]
  [socCell5] -> socCellMux/5
  Module5_outputs/4 -> [socCell5]
  [numCycles5] -> numCyclesMux/5
  Module5_outputs/3 -> [numCycles5]
  [batteryVoltage5] -> batteryVoltageMux/5
  Module5_outputs/2 -> [batteryVoltage5]
  [batteryCurrent5] -> batteryCurrentMux/5
  Module5_outputs/1 -> [batteryCurrent5]
  [vParallelAssembly4] -> vParallelAssemblyMux/4
  Module4_outputs/6 -> [vParallelAssembly4]
  [socParallelAssembly4] -> socParallelAssemblyMux/4
  Module4_outputs/5 -> [socParallelAssembly4]
  [socCell4] -> socCellMux/4
  Module4_outputs/4 -> [socCell4]
  [numCycles4] -> numCyclesMux/4
  Module4_outputs/3 -> [numCycles4]
  [batteryVoltage4] -> batteryVoltageMux/4
  Module4_outputs/2 -> [batteryVoltage4]
  [batteryCurrent4] -> batteryCurrentMux/4
  Module4_outputs/1 -> [batteryCurrent4]
  [vParallelAssembly3] -> vParallelAssemblyMux/3
  Module3_outputs/6 -> [vParallelAssembly3]
  [socParallelAssembly3] -> socParallelAssemblyMux/3
  Module3_outputs/5 -> [socParallelAssembly3]
  [socCell3] -> socCellMux/3
  Module3_outputs/4 -> [socCell3]
  [numCycles3] -> numCyclesMux/3
  Module3_outputs/3 -> [numCycles3]
  [batteryVoltage3] -> batteryVoltageMux/3
  Module3_outputs/2 -> [batteryVoltage3]
  [batteryCurrent3] -> batteryCurrentMux/3
  Module3_outputs/1 -> [batteryCurrent3]
  [vParallelAssembly2] -> vParallelAssemblyMux/2
  Module2_outputs/6 -> [vParallelAssembly2]
  [socParallelAssembly2] -> socParallelAssemblyMux/2
  Module2_outputs/5 -> [socParallelAssembly2]
  [socCell2] -> socCellMux/2
  Module2_outputs/4 -> [socCell2]
  [numCycles2] -> numCyclesMux/2
  Module2_outputs/3 -> [numCycles2]
  [batteryVoltage2] -> batteryVoltageMux/2
  Module2_outputs/2 -> [batteryVoltage2]
  [batteryCurrent2] -> batteryCurrentMux/2
  Module2_outputs/1 -> [batteryCurrent2]
  [vParallelAssembly1] -> vParallelAssemblyMux/1
  vParallelAssemblyMux/1 -> vParallelAssembly/1
  Segment_outputs/6 -> [vParallelAssembly1]
  [socParallelAssembly1] -> socParallelAssemblyMux/1
  socParallelAssemblyMux/1 -> socParallelAssembly/1
  Segment_outputs/5 -> [socParallelAssembly1]
  [socCell1] -> socCellMux/1
  socCellMux/1 -> socCell/1
  Segment_outputs/4 -> [socCell1]
  [numCycles1] -> numCyclesMux/1
  numCyclesMux/1 -> numCycles/1
  Segment_outputs/3 -> [numCycles1]
  [batteryVoltage1] -> batteryVoltageMux/1
  batteryVoltageMux/1 -> batteryVoltage/1
  Segment_outputs/2 -> [batteryVoltage1]
  [batteryCurrent1] -> batteryCurrentMux/1
  batteryCurrentMux/1 -> batteryCurrent/1
  Segment_outputs/1 -> [batteryCurrent1]
  connections:
  Module5/RConn1 -- -/RConn1
  Segment/LConn1 -- +/RConn1
  Module5/LConn1 -- Module4/RConn1
  Module4/LConn1 -- Module3/RConn1
  Module3/LConn1 -- Module2/RConn1
  Module2/LConn1 -- Segment/RConn1
